simulink model "mpc1_p2"  (R2023a)
settings: Solver=FixedStepDiscrete  StartTime=0.0  StopTime=100  FixedStep=0.5  RelTol=1e-3
libraries: mpclib x1, cstblocks x1
settings Model: Creator=z92504901  LastModifiedBy=z92504194

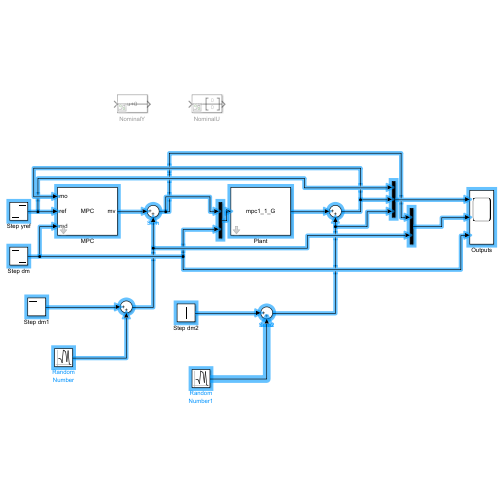
[thumbnail: Simulink's stored preview of the top-level diagram]
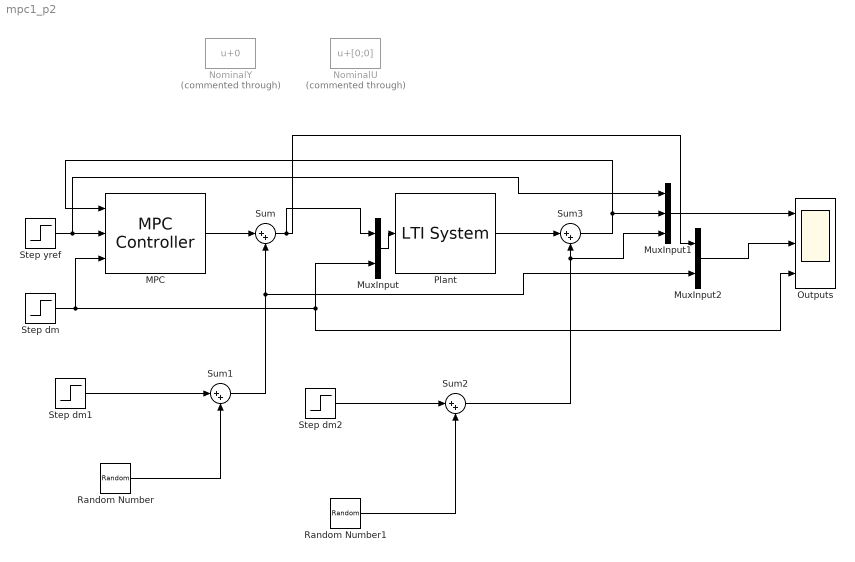
== system mpc1_p2 ==
  MPC : mpclib/MPC Controller  SCDEnableBlockLinearizationSpecification=on  mpcobj=mpc1_1_C  is_multiple=0  enable_value=0  return_u0=off  updateMPCinCallerWorkspace=on  md_inport=on  mv_inport=off  uref_inport=off  return_cost=off  return_mvseq=off  return_qpstatus=off  return_xseq=off  return_state=off  return_ovseq=off  state_inport=off  umin_inport=off  umax_inport=off  ymin_inport=off  ymax_inport=off  cc_inport=off  ywt_inport=off  uwt_inport=off  duwt_inport=off  rhoeps_inport=off  pm_inport=off  MaximumP=10  HorizonChoice=FixedHorizon  n_ts=0.5  n_p=10  n_mv=1  n_md=1  n_ud=0  n_mo=1  n_uo=0  BlockDataType=double  SampleTimeInherited=off  switch_inport=off
  MuxInput : Mux  Inputs=2
  MuxInput1 : Mux  Inputs=3
  MuxInput2 : Mux  Inputs=2
  NominalU : Bias  Commented=through  Bias=[0;0]
  NominalY : Bias  Commented=through
  Outputs : Scope  NumInputPorts=3
  Plant : cstblocks/LTI System  sys=mpc1_1_G  IC=[]
  Random Number : RandomNumber  Variance=0.0001  SampleTime=0.5
  Random Number1 : RandomNumber  Variance=0.0001  SampleTime=0.5
  Step dm : Step  Time=20  After=-5
  Step dm1 : Step  Time=50  After=-0.1
  Step dm2 : Step  Time=30
  Step yref : Step  Time=10  After=20
  Sum{,1..3} (4 alike) : Sum  Inputs=|++
  wires:
  Step yref/1 -> MuxInput1/1, MPC/2
  MPC/1 -> Sum/1
  Step dm/1 -> MuxInput/2, Outputs/3, MPC/3
  MuxInput/1 -> Plant/1
  MuxInput1/1 -> Outputs/1
  Sum1/1 -> MuxInput2/2, Sum/2
  Step dm1/1 -> Sum1/1
  Random Number/1 -> Sum1/2
  Random Number1/1 -> Sum2/2
  Step dm2/1 -> Sum2/1
  Plant/1 -> Sum3/1
  Sum2/1 -> MuxInput1/3, Sum3/2
  Sum3/1 -> MPC/1, MuxInput1/2
  MuxInput2/1 -> Outputs/2
  Sum/1 -> MuxInput/1, MuxInput2/1
